simulink model "scheme_L2"  (R2025b)
settings: Solver=ode45  StartTime=0.0  StopTime=10  MaxStep=0.005  RelTol=1e-3
settings Model: Creator=Alexandr  LastModifiedBy=Alexandr

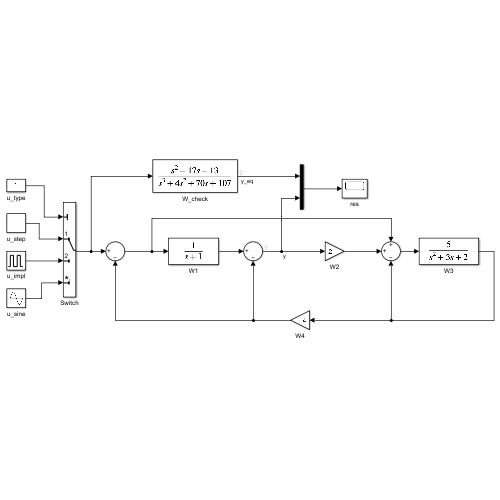
[thumbnail: Simulink's stored preview of the top-level diagram]
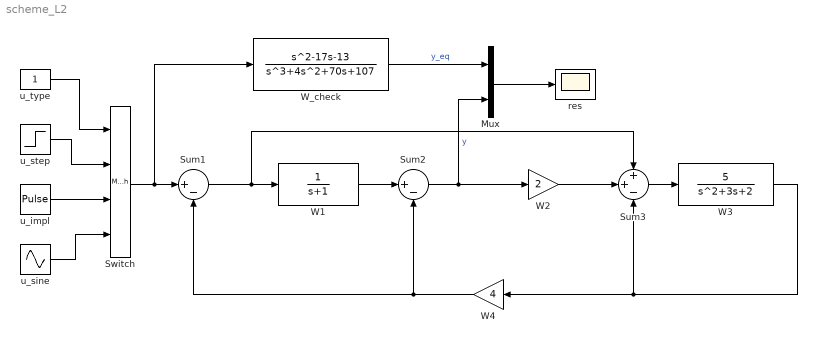
== system scheme_L2 ==
  Mux : Mux  Inputs=2
  Sum1 : Sum  Inputs=|+-
  Sum2 : Sum  Inputs=|+-
  Sum3 : Sum  Inputs=++-
  Switch : MultiPortSwitch  SaturateOnIntegerOverflow=off  InputSameDT=off
  W1 : TransferFcn  Denominator=[1 1]
  W2 : Gain  Gain=2
  W3 : TransferFcn  Numerator=[5]  Denominator=[1 3 2]
  W4 : Gain  Gain=4
  W_check : TransferFcn  Numerator=[1 -17 -13]  Denominator=[1 4 70 107]
  res : Scope
  u_impl : DiscretePulseGenerator  PulseType=Time based  Amplitude=20  Period=20  PulseWidth=0.2  PhaseDelay=2
  u_sine : Sin  Frequency=3  SampleTime=0
  u_step : Step  SampleTime=0
  u_type : Constant
  wires:
  W1/1 -> Sum2/1
  W_check/1 -> Mux/1  "y_eq"
  u_type/1 -> Switch/1
  u_step/1 -> Switch/2
  u_impl/1 -> Switch/3
  u_sine/1 -> Switch/4
  Switch/1 -> W_check/1, Sum1/1
  Sum2/1 -> W2/1, Mux/2  "y"
  Sum1/1 -> Sum3/1, W1/1
  W4/1 -> Sum1/2, Sum2/2
  Mux/1 -> res/1
  W2/1 -> Sum3/2
  W3/1 -> Sum3/3, W4/1
  Sum3/1 -> W3/1
